simulink model "nms_sim_2D_cost"  (R2024b)
settings: Solver=ode15s  StartTime=0.0  StopTime=t_sim  MaxStep=dt_max  EnableMultiTasking=on
values from neighbouring files (symbols this model uses):
  a_BFSH = param_ctrl(35)*1    [setCtrlPar_optim_CPGreflex2001_2D.m]
  a_GAS = param_ctrl(37)*1    [setCtrlPar_optim_CPGreflex2001_2D.m]
  a_GLU = param_ctrl(31)*1    [setCtrlPar_optim_CPGreflex2001_2D.m]
  a_HAM = param_ctrl(33)*1    [setCtrlPar_optim_CPGreflex2001_2D.m]
  a_HFL = param_ctrl(32)*1    [setCtrlPar_optim_CPGreflex2001_2D.m]
  a_RF = param_ctrl(34)*1    [setCtrlPar_optim_CPGreflex2001_2D.m]
  a_SOL = param_ctrl(38)*1    [setCtrlPar_optim_CPGreflex2001_2D.m]
  a_TA = param_ctrl(39)*1    [setCtrlPar_optim_CPGreflex2001_2D.m]
  a_VAS = param_ctrl(36)*1    [setCtrlPar_optim_CPGreflex2001_2D.m]
  ai = param_ctrl(96)*2.0    [setCtrlPar_optim_CPGreflex2001_2D.m]
  b_BFSH = param_ctrl(52)*.51    [setCtrlPar_optim_CPGreflex2001_2D.m]
  b_BFSHGAS = param_ctrl(55)*.51    [setCtrlPar_optim_CPGreflex2001_2D.m]
  b_BFSHHAM = param_ctrl(54)*.51    [setCtrlPar_optim_CPGreflex2001_2D.m]
  b_BFSHVAS = param_ctrl(53)*.51    [setCtrlPar_optim_CPGreflex2001_2D.m]
  b_GAS = param_ctrl(59)*.51    [setCtrlPar_optim_CPGreflex2001_2D.m]
  b_GASBFSH = param_ctrl(60)*.51    [setCtrlPar_optim_CPGreflex2001_2D.m]
  b_GASSOL = param_ctrl(61)*.51    [setCtrlPar_optim_CPGreflex2001_2D.m]
  b_GLU = param_ctrl(40)*.51    [setCtrlPar_optim_CPGreflex2001_2D.m]
  b_GLUHAM = param_ctrl(42)*.51    [setCtrlPar_optim_CPGreflex2001_2D.m]
  b_GLUHFL = param_ctrl(41)*.51    [setCtrlPar_optim_CPGreflex2001_2D.m]
  b_HAM = param_ctrl(46)*.51    [setCtrlPar_optim_CPGreflex2001_2D.m]
  b_HAMBFSH = param_ctrl(48)*.51    [setCtrlPar_optim_CPGreflex2001_2D.m]
  b_HAMGLU = param_ctrl(47)*.51    [setCtrlPar_optim_CPGreflex2001_2D.m]
  b_HFL = param_ctrl(43)*.51    [setCtrlPar_optim_CPGreflex2001_2D.m]
  b_HFLGLU = param_ctrl(44)*.51    [setCtrlPar_optim_CPGreflex2001_2D.m]
  b_HFLRF = param_ctrl(45)*.51    [setCtrlPar_optim_CPGreflex2001_2D.m]
  b_RF = param_ctrl(49)*.51    [setCtrlPar_optim_CPGreflex2001_2D.m]
  b_RFHFL = param_ctrl(50)*.51    [setCtrlPar_optim_CPGreflex2001_2D.m]
  b_RFVAS = param_ctrl(51)*.51    [setCtrlPar_optim_CPGreflex2001_2D.m]
  b_SOL = param_ctrl(62)*.51    [setCtrlPar_optim_CPGreflex2001_2D.m]
  b_SOLGAS = param_ctrl(64)*.51    [setCtrlPar_optim_CPGreflex2001_2D.m]
  b_SOLTA = param_ctrl(63)*.51    [setCtrlPar_optim_CPGreflex2001_2D.m]
  b_TA = param_ctrl(65)*.51    [setCtrlPar_optim_CPGreflex2001_2D.m]
  b_TASOL = param_ctrl(66)*.51    [setCtrlPar_optim_CPGreflex2001_2D.m]
  b_VAS = param_ctrl(56)*.51    [setCtrlPar_optim_CPGreflex2001_2D.m]
  b_VASBFSH = param_ctrl(57)*.51    [setCtrlPar_optim_CPGreflex2001_2D.m]
  b_VASRF = param_ctrl(58)*.51    [setCtrlPar_optim_CPGreflex2001_2D.m]
  bias = param_ctrl(97)*2.5    [setCtrlPar_optim_CPGreflex2001_2D.m]
  c = 0.05    [nms_MS_2D_scaled.m]
  c_jointstop = 0.3 / (pi/180)    (= 17.1887338539)    [nms_MS_2D_scaled.m]
  D12_F = 0.16    *scaleL_JPhys    [nms_MechInit_2D_scaleSkel.m]
  D12_S = 0.2460	*sub_height    [nms_MechInit_2D_scaleSkel.m]
  D12_T = 0.2450  *sub_height    [nms_MechInit_2D_scaleSkel.m]
  D12y_F = 0.039  *sub_height    [nms_MechInit_2D_scaleSkel.m]
  D12z_HAT = 0.1    [nms_MS_2D_scaled.m]
  D13_F = 0.20    *scaleL_JPhys    [nms_MechInit_2D_scaleSkel.m]
  D1G_F = 0.14    *scaleL_JPhys    [nms_MechInit_2D_scaleSkel.m]
  D1G_HAT = 0.35  *scaleL_JPhys    [nms_MechInit_2D_scaleSkel.m]
  D1G_S = (0.3 - D12y_F/4)	*scaleL_JPhys    [nms_MechInit_2D_scaleSkel.m]
  D1G_T = (0.3 - D12y_F/4)	*scaleL_JPhys    [nms_MechInit_2D_scaleSkel.m]
  D1Gy_F = D12y_F*D1G_F/D12_F    (= 0.07)    [nms_MechInit_2D_scaleSkel.m]
  d_BFSH = param_ctrl(26)*1    [setCtrlPar_optim_CPGreflex2001_2D.m]
  d_GAS = param_ctrl(28)*1    [setCtrlPar_optim_CPGreflex2001_2D.m]
  d_GLU = param_ctrl(22)*1    [setCtrlPar_optim_CPGreflex2001_2D.m]
  d_HAM = param_ctrl(24)*1    [setCtrlPar_optim_CPGreflex2001_2D.m]
  d_HFL = param_ctrl(23)*1    [setCtrlPar_optim_CPGreflex2001_2D.m]
  d_RF = param_ctrl(25)*1    [setCtrlPar_optim_CPGreflex2001_2D.m]
  d_SOL = param_ctrl(29)*1    [setCtrlPar_optim_CPGreflex2001_2D.m]
  d_TA = param_ctrl(30)*1    [setCtrlPar_optim_CPGreflex2001_2D.m]
  d_VAS = param_ctrl(27)*1    [setCtrlPar_optim_CPGreflex2001_2D.m]
  DeltaThRef = 5e-3    (= 0.005)    [nms_MS_2D_scaled.m]
  dloptBFSH = 3.0    (= 3)    [setCtrlPar_optim_CPGreflex2001_2D.m]
  dloptGAS = 3.0    (= 3)    [setCtrlPar_optim_CPGreflex2001_2D.m]
  dloptGLU = 3.0    (= 3)    [setCtrlPar_optim_CPGreflex2001_2D.m]
  dloptHAM = 3.0    (= 3)    [setCtrlPar_optim_CPGreflex2001_2D.m]
  dloptHFL = 3.0    (= 3)    [setCtrlPar_optim_CPGreflex2001_2D.m]
  dloptRF = 3.0    (= 3)    [setCtrlPar_optim_CPGreflex2001_2D.m]
  dloptSOL = 3.0    (= 3)    [setCtrlPar_optim_CPGreflex2001_2D.m]
  dloptTA = 3.0    (= 3)    [setCtrlPar_optim_CPGreflex2001_2D.m]
  dloptVAS = 3.0    (= 3)    [setCtrlPar_optim_CPGreflex2001_2D.m]
  ec_BFSH = param_ctrl(80)*0.15    [setCtrlPar_optim_CPGreflex2001_2D.m]
  ec_GAS = param_ctrl(82)*0.15    [setCtrlPar_optim_CPGreflex2001_2D.m]
  ec_GLU = param_ctrl(76)*0.15    [setCtrlPar_optim_CPGreflex2001_2D.m]
  ec_HAM = param_ctrl(78)*0.15    [setCtrlPar_optim_CPGreflex2001_2D.m]
  ec_HFL = param_ctrl(77)*0.15    [setCtrlPar_optim_CPGreflex2001_2D.m]
  ec_RF = param_ctrl(79)*0.15    [setCtrlPar_optim_CPGreflex2001_2D.m]
  ec_TA = param_ctrl(84)*0.15    [setCtrlPar_optim_CPGreflex2001_2D.m]
  ec_VAS = param_ctrl(81)*0.15    [setCtrlPar_optim_CPGreflex2001_2D.m]
  eref = 0.04    [nms_MS_2D_scaled.m]
  eref_GAS = 0.1    [nms_MS_2D_scaled.m]
  eref_SOL = 0.1    [nms_MS_2D_scaled.m]
  es_BFSH = param_ctrl(89)*0.15    [setCtrlPar_optim_CPGreflex2001_2D.m]
  es_GAS = param_ctrl(91)*0.15    [setCtrlPar_optim_CPGreflex2001_2D.m]
  es_GLU = param_ctrl(85)*0.15    [setCtrlPar_optim_CPGreflex2001_2D.m]
  es_HAM = param_ctrl(87)*0.15    [setCtrlPar_optim_CPGreflex2001_2D.m]
  es_HFL = param_ctrl(86)*0.15    [setCtrlPar_optim_CPGreflex2001_2D.m]
  es_RF = param_ctrl(88)*0.15    [setCtrlPar_optim_CPGreflex2001_2D.m]
  es_TA = param_ctrl(93)*0.15    [setCtrlPar_optim_CPGreflex2001_2D.m]
  es_VAS = param_ctrl(90)*0.15    [setCtrlPar_optim_CPGreflex2001_2D.m]
  FmaxBFSH = 350    [nms_MS_2D_scaled.m]
  FmaxGAS = 2000    [nms_MS_2D_scaled.m]
  FmaxGLU = 4000    [nms_MS_2D_scaled.m]
  FmaxHAM = 2000    [nms_MS_2D_scaled.m]
  FmaxHFL = 2000    [nms_MS_2D_scaled.m]
  FmaxRF = 850    [nms_MS_2D_scaled.m]
  FmaxSOL = 4000    [nms_MS_2D_scaled.m]
  FmaxTA = 800    [nms_MS_2D_scaled.m]
  FmaxVAS = 5000    [nms_MS_2D_scaled.m]
  g = 9.81    [nms_MS_2D_scaled.m]
  gamma_4 = param_ctrl(11) * 1.7    [setCtrlPar_optim_CPGreflexsynergy2023_2D.m]
  h_BFSH = param_ctrl(71)*.1    [setCtrlPar_optim_CPGreflex2001_2D.m]
  h_GAS = param_ctrl(73)*.1    [setCtrlPar_optim_CPGreflex2001_2D.m]
  h_GLU = param_ctrl(67)*.1    [setCtrlPar_optim_CPGreflex2001_2D.m]
  h_HAM = param_ctrl(69)*.1    [setCtrlPar_optim_CPGreflex2001_2D.m]
  h_HFL = param_ctrl(68)*.1    [setCtrlPar_optim_CPGreflex2001_2D.m]
  h_RF = param_ctrl(70)*.1    [setCtrlPar_optim_CPGreflex2001_2D.m]
  h_SOL = param_ctrl(74)*.1    [setCtrlPar_optim_CPGreflex2001_2D.m]
  h_TA = param_ctrl(75)*.1    [setCtrlPar_optim_CPGreflex2001_2D.m]
  h_VAS = param_ctrl(72)*.1    [setCtrlPar_optim_CPGreflex2001_2D.m]
  HLCtrlPar = [theta_tgt l_clr alpha_tgt alpha_cd alpha_cv]    [setCtrlPar_optim_reflex2015_2D.m]
  In_F = 0.005    *scaleM*scaleL_JPhys^2    [nms_MechInit_2D_scaleSkel.m]
  In_HAT = 2.5    *scaleM*scaleL_JPhys^2    [nms_MechInit_2D_scaleSkel.m]
  In_S = 0.05     *scaleM*scaleL_JPhys^2    [nms_MechInit_2D_scaleSkel.m]
  In_T = 0.15     *scaleM*scaleL_JPhys^2    [nms_MechInit_2D_scaleSkel.m]
  init_exc = 0.01    [setInitPar_optim_2D.m]
  init_fm = 0.01    [setInitPar_optim_2D.m]
  init_lce = 1    [setInitPar_optim_2D.m]
  init_LCPG = param_ctrl(12) * 0.01    [setCtrlPar_optim_CPGreflexsynergy2023_2D.m]
  init_LStance = 1    [setInitPar_optim_2D.m]
  init_N1 = osc_signal1(phi_off_osc_ind)    [setCtrlPar_optim_CPGreflex2001_2D.m]
  ... (+441 more)
undefined symbols (not defined in the file or in its folder): cost_act_exponent, cost_v_tgt, flag_controller, Newton, nStep_obj, nStep_startKin, Raphson, sgn, SSW_kin, terrain_slope_angle, v_plateS1, X, Y, Z
libraries: nesl_utility x94, sm_lib x90, simulink x28, simulink_extras x12
(part 9 of 20)

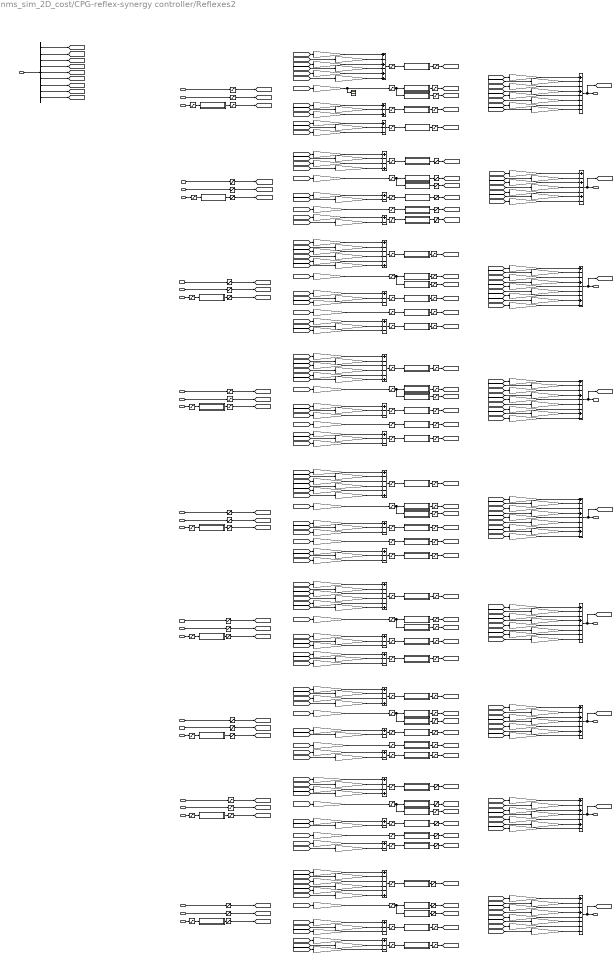
== system nms_sim_2D_cost/CPG-reflex-synergy controller/Reflexes2 ==
  note: GLU
  note: Sensory Neurons
  note: Inter Neurons
  note: Reflex output to Motoneurons
  note: HFL
  note: HAM
  note: RF
  note: VAS
  note: BFSH
  note: GAS
  note: SOL
  note: TA
  note: Muscle Activations (MN) RC
  FmGLU : Inport
  LceGLU : Inport  Port=2
  VceGLU : Inport  Port=3
  FmHFL : Inport  Port=4
  LceHFL : Inport  Port=5
  VceHFL : Inport  Port=6
  FmHAM : Inport  Port=7
  LceHAM : Inport  Port=8
  VceHAM : Inport  Port=9
  FmRF : Inport  Port=10
  LceRF : Inport  Port=11
  VceRF : Inport  Port=12
  FmVAS : Inport  Port=13
  LceVAS : Inport  Port=14
  VceVAS : Inport  Port=15
  FmBFSH : Inport  Port=16
  LceBFSH : Inport  Port=17
  VceBFSH : Inport  Port=18
  FmGAS : Inport  Port=19
  LceGAS : Inport  Port=20
  VceGAS : Inport  Port=21
  FmSOL : Inport  Port=22
  LceSOL : Inport  Port=23
  VceSOL : Inport  Port=24
  FmTA : Inport  Port=25
  LceTA : Inport  Port=26
  VceTA : Inport  Port=27
  Act : Inport  Port=28
  Demux : Demux  Outputs=9
  Gain1 : Gain  Gain=k_INIA_HFL_SNIA_HFL
  Gain10 : Gain  Gain=k_INIB_HFL_INIB_HAM
  Gain100 : Gain  Gain=k_INIA_TA_INIA_GAS
  Gain101 : Gain  Gain=k_INIA_TA_INIA_SOL
  Gain102 : Gain  Gain=k_INIA_TA_INRC_GAS
  Gain103 : Gain  Gain=k_INIA_TA_INRC_SOL
  Gain104 : Gain  Gain=k_INIA_TA_MN_TA
  Gain105 : Gain  Gain=k_INII_TA_SNII_TA
  Gain106 : Gain  Gain=k_INIB_TA_SNIB_TA
  Gain107 : Gain  Gain=k_INIB_TA_INIB_GAS
  Gain108 : Gain  Gain=k_INIB_TA_INIB_SOL
  Gain109 : Gain  Gain=k_INRC_TA_Act_TA
  Gain11 : Gain  Gain=k_INRC_HFL_INRC_HAM
  Gain110 : Gain  Gain=k_INRC_TA_INRC_GAS
  Gain111 : Gain  Gain=k_INRC_TA_INRC_SOL
  Gain112 : Gain  Gain=k_MN_HFL_SNIA_HFL
  Gain113 : Gain  Gain=k_MN_HFL_INIA_GLU
  Gain114 : Gain  Gain=k_MN_HFL_INIA_HAM
  Gain115 : Gain  Gain=k_MN_HFL_INII_HFL
  Gain116 : Gain  Gain=k_MN_HFL_INII_GLU
  Gain117 : Gain  Gain=k_MN_HFL_INII_HAM
  Gain118 : Gain  Gain=k_MN_HFL_INIB_HFL
  Gain119 : Gain  Gain=k_MN_HFL_INRC_HFL
  Gain12 : Gain  Gain=k_INRC_HFL_Act_HFL
  Gain120 : Gain  Gain=k_MN_GLU_SNIA_GLU
  Gain121 : Gain  Gain=k_MN_GLU_INIA_HFL
  Gain122 : Gain  Gain=k_MN_GLU_INII_GLU
  Gain123 : Gain  Gain=k_MN_GLU_INII_HFL
  Gain124 : Gain  Gain=k_MN_GLU_INIB_GLU
  Gain125 : Gain  Gain=k_MN_GLU_INIBext_GLU
  Gain126 : Gain  Gain=k_MN_GLU_INRC_GLU
  Gain127 : Gain  Gain=k_MN_HAM_SNIA_HAM
  Gain128 : Gain  Gain=k_MN_HAM_INIA_VAS
  Gain129 : Gain  Gain=k_MN_HAM_INIA_RF
  Gain13 : Gain  Gain=k_INRC_HFL_INRC_GLU
  Gain130 : Gain  Gain=k_MN_HAM_INII_HAM
  Gain131 : Gain  Gain=k_MN_HAM_INII_VAS
  Gain132 : Gain  Gain=k_MN_HAM_INII_RF
  Gain133 : Gain  Gain=k_MN_HAM_INIB_HAM
  Gain134 : Gain  Gain=k_MN_HAM_INIBext_HAM
  Gain135 : Gain  Gain=k_MN_HAM_INRC_HAM
  Gain136 : Gain  Gain=k_MN_RF_SNIA_RF
  Gain137 : Gain  Gain=k_MN_RF_INIA_HAM
  Gain138 : Gain  Gain=k_MN_RF_INIA_BFSH
  Gain139 : Gain  Gain=k_MN_RF_INII_RF
  Gain14 : Gain  Gain=k_INIA_GLU_INRC_HFL
  Gain140 : Gain  Gain=k_MN_RF_INII_HAM
  Gain141 : Gain  Gain=k_MN_RF_INII_BFSH
  Gain142 : Gain  Gain=k_MN_RF_INIB_RF
  Gain143 : Gain  Gain=k_MN_RF_INIBext_RF
  Gain144 : Gain  Gain=k_MN_RF_INRC_RF
  Gain145 : Gain  Gain=k_MN_VAS_SNIA_VAS
  Gain146 : Gain  Gain=k_MN_VAS_INIA_HAM
  Gain147 : Gain  Gain=k_MN_VAS_INIA_BFSH
  Gain148 : Gain  Gain=k_MN_VAS_INII_VAS
  Gain149 : Gain  Gain=k_MN_VAS_INII_HAM
  Gain15 : Gain  Gain=k_INIA_GLU_SNIA_GLU
  Gain150 : Gain  Gain=k_MN_VAS_INII_BFSH
  Gain151 : Gain  Gain=k_MN_VAS_INIB_VAS
  Gain152 : Gain  Gain=k_MN_VAS_INIBext_VAS
  Gain153 : Gain  Gain=k_MN_VAS_INRC_VAS
  Gain154 : Gain  Gain=k_MN_BFSH_SNIA_BFSH
  Gain155 : Gain  Gain=k_MN_BFSH_INIA_VAS
  Gain156 : Gain  Gain=k_MN_BFSH_INIA_RF
  Gain157 : Gain  Gain=k_MN_BFSH_INII_BFSH
  Gain158 : Gain  Gain=k_MN_BFSH_INII_VAS
  Gain159 : Gain  Gain=k_MN_BFSH_INII_RF
  Gain16 : Gain  Gain=k_INIA_GLU_INIA_HFL
  Gain160 : Gain  Gain=k_MN_BFSH_INIB_BFSH
  Gain161 : Gain  Gain=k_MN_BFSH_INRC_BFSH
  Gain162 : Gain  Gain=k_MN_GAS_SNIA_GAS
  Gain163 : Gain  Gain=k_MN_GAS_INIA_TA
  Gain164 : Gain  Gain=k_MN_GAS_INII_GAS
  Gain165 : Gain  Gain=k_MN_GAS_INII_TA
  Gain166 : Gain  Gain=k_MN_GAS_INIB_GAS
  Gain167 : Gain  Gain=k_MN_GAS_INIBext_GAS
  Gain168 : Gain  Gain=k_MN_GAS_INRC_GAS
  Gain169 : Gain  Gain=k_MN_SOL_SNIA_SOL
  Gain17 : Gain  Gain=k_INIA_GLU_MN_GLU
  Gain170 : Gain  Gain=k_MN_SOL_INIA_TA
  Gain171 : Gain  Gain=k_MN_SOL_INII_SOL
  Gain172 : Gain  Gain=k_MN_SOL_INII_TA
  Gain173 : Gain  Gain=k_MN_SOL_INIB_SOL
  Gain174 : Gain  Gain=k_MN_SOL_INIBext_SOL
  Gain175 : Gain  Gain=k_MN_SOL_INRC_SOL
  Gain176 : Gain  Gain=k_MN_TA_SNIA_TA
  Gain177 : Gain  Gain=k_MN_TA_INIA_GAS
  Gain178 : Gain  Gain=k_MN_TA_INIA_SOL
  Gain179 : Gain  Gain=k_MN_TA_INII_TA
  Gain18 : Gain  Gain=k_INII_GLU_SNII_GLU
  Gain180 : Gain  Gain=k_MN_TA_INII_GAS
  Gain181 : Gain  Gain=k_MN_TA_INII_SOL
  Gain182 : Gain  Gain=k_MN_TA_INIB_TA
  Gain183 : Gain  Gain=k_MN_TA_INRC_TA
  Gain19 : Gain  Gain=k_INIB_GLU_SNIB_GLU
  Gain2 : Gain  Gain=k_INIA_HFL_INIA_GLU
  Gain20 : Gain  Gain=k_INIB_GLU_INIB_HFL
  Gain21 : Gain  Gain=k_INIB_GLU_SNIBext_GLU
  Gain22 : Gain  Gain=k_INRC_GLU_Act_GLU
  Gain23 : Gain  Gain=k_INRC_GLU_INRC_HFL
  Gain24 : Gain  Gain=k_INIA_HAM_SNIA_HAM
  Gain25 : Gain  Gain=k_INIA_HAM_INIA_VAS
  Gain26 : Gain  Gain=k_INIA_HAM_INIA_RF
  Gain27 : Gain  Gain=k_INIA_HAM_INRC_VAS
  Gain28 : Gain  Gain=k_INIA_HAM_INRC_RF
  Gain29 : Gain  Gain=k_INIA_HAM_MN_HAM
  Gain3 : Gain  Gain=k_INIA_HFL_INIA_HAM
  Gain30 : Gain  Gain=k_INII_HAM_SNII_HAM
  Gain31 : Gain  Gain=k_INIB_HAM_SNIB_HAM
  Gain32 : Gain  Gain=k_INIB_HAM_INIB_VAS
  Gain33 : Gain  Gain=k_INIB_HAM_INIB_RF
  Gain34 : Gain  Gain=k_INIB_HAM_SNIBext_HAM
  Gain35 : Gain  Gain=k_INRC_HAM_Act_HAM
  Gain36 : Gain  Gain=k_INRC_HAM_INRC_VAS
  Gain37 : Gain  Gain=k_INRC_HAM_INRC_RF
  Gain38 : Gain  Gain=k_INIA_RF_SNIA_RF
  Gain39 : Gain  Gain=k_INIA_RF_INIA_HAM
  Gain4 : Gain  Gain=k_INIA_HFL_INRC_GLU
  Gain40 : Gain  Gain=k_INIA_RF_INIA_BFSH
  Gain41 : Gain  Gain=k_INIA_RF_INRC_HAM
  Gain42 : Gain  Gain=k_INIA_RF_INRC_BFSH
  Gain43 : Gain  Gain=k_INIA_RF_MN_RF
  Gain44 : Gain  Gain=k_INII_RF_SNII_RF
  Gain45 : Gain  Gain=k_INIB_RF_SNIB_RF
  Gain46 : Gain  Gain=k_INIB_RF_INIB_HAM
  Gain47 : Gain  Gain=k_INIB_RF_INIB_BFSH
  Gain48 : Gain  Gain=k_INIB_RF_SNIBext_RF
  Gain49 : Gain  Gain=k_INRC_RF_Act_RF
  Gain5 : Gain  Gain=k_INIA_HFL_INRC_HAM
  Gain50 : Gain  Gain=k_INRC_RF_INRC_HAM
  Gain51 : Gain  Gain=k_INRC_RF_INRC_BFSH
  Gain52 : Gain  Gain=k_INIA_VAS_SNIA_VAS
  Gain53 : Gain  Gain=k_INIA_VAS_INIA_HAM
  Gain54 : Gain  Gain=k_INIA_VAS_INIA_BFSH
  Gain55 : Gain  Gain=k_INIA_VAS_INRC_HAM
  Gain56 : Gain  Gain=k_INIA_VAS_INRC_BFSH
  Gain57 : Gain  Gain=k_INIA_VAS_MN_VAS
  Gain58 : Gain  Gain=k_INII_VAS_SNII_VAS
  Gain59 : Gain  Gain=k_INIB_VAS_SNIB_VAS
  Gain6 : Gain  Gain=k_INII_HFL_SNII_HFL
  Gain60 : Gain  Gain=k_INIB_VAS_INIB_HAM
  Gain61 : Gain  Gain=k_INIB_VAS_INIB_BFSH
  Gain62 : Gain  Gain=k_INRC_VAS_Act_VAS
  Gain63 : Gain  Gain=k_INRC_VAS_INRC_HAM
  Gain64 : Gain  Gain=k_INRC_VAS_INRC_BFSH
  Gain65 : Gain  Gain=k_INIB_VAS_SNIBext_VAS
  Gain66 : Gain  Gain=k_INIA_BFSH_SNIA_BFSH
  Gain67 : Gain  Gain=k_INIA_BFSH_INIA_VAS
  Gain68 : Gain  Gain=k_INIA_BFSH_INIA_RF
  Gain69 : Gain  Gain=k_INIA_BFSH_INRC_VAS
  Gain7 : Gain  Gain=k_INIA_HFL_MN_HFL
  Gain70 : Gain  Gain=k_INIA_BFSH_INRC_RF
  Gain71 : Gain  Gain=k_INIA_BFSH_MN_BFSH
  Gain72 : Gain  Gain=k_INII_BFSH_SNII_BFSH
  Gain73 : Gain  Gain=k_INIB_BFSH_SNIB_BFSH
  Gain74 : Gain  Gain=k_INIB_BFSH_INIB_VAS
  Gain75 : Gain  Gain=k_INIB_BFSH_INIB_RF
  Gain76 : Gain  Gain=k_INRC_BFSH_Act_BFSH
  Gain77 : Gain  Gain=k_INRC_BFSH_INRC_VAS
  Gain78 : Gain  Gain=k_INRC_BFSH_INRC_RF
  Gain79 : Gain  Gain=k_INIA_GAS_SNIA_GAS
  Gain8 : Gain  Gain=k_INIB_HFL_SNIB_HFL
  Gain80 : Gain  Gain=k_INIA_GAS_INIA_TA
  Gain81 : Gain  Gain=k_INIA_GAS_INRC_TA
  Gain82 : Gain  Gain=k_INIA_GAS_MN_GAS
  Gain83 : Gain  Gain=k_INII_GAS_SNII_GAS
  Gain84 : Gain  Gain=k_INIB_GAS_SNIB_GAS
  Gain85 : Gain  Gain=k_INIB_GAS_INIB_TA
  Gain86 : Gain  Gain=k_INRC_GAS_Act_GAS
  Gain87 : Gain  Gain=k_INRC_GAS_INRC_TA
  Gain88 : Gain  Gain=k_INIB_GAS_SNIBext_GAS
  Gain89 : Gain  Gain=k_INIA_SOL_SNIA_SOL
  Gain9 : Gain  Gain=k_INIB_HFL_INIB_GLU
  Gain90 : Gain  Gain=k_INIA_SOL_INIA_TA
  Gain91 : Gain  Gain=k_INIA_SOL_INRC_TA
  Gain92 : Gain  Gain=k_INIA_SOL_MN_SOL
  Gain93 : Gain  Gain=k_INII_SOL_SNII_SOL
  Gain94 : Gain  Gain=k_INIB_SOL_SNIB_SOL
  Gain95 : Gain  Gain=k_INIB_SOL_INIB_TA
  Gain96 : Gain  Gain=k_INIB_SOL_SNIBext_SOL
  Gain97 : Gain  Gain=k_INRC_SOL_Act_SOL
  Gain98 : Gain  Gain=k_INRC_SOL_INRC_TA
  Gain99 : Gain  Gain=k_INIA_TA_SNIA_TA
  IN RC1 : Subsystem
  IN RC10 : Subsystem
  IN RC11 : Subsystem
  IN RC12 : Subsystem
  IN RC13 : Subsystem
  IN RC14 : Subsystem
  IN RC15 : Subsystem
  IN RC16 : Subsystem
  IN RC17 : Subsystem
  IN RC18 : Subsystem
  IN RC19 : Subsystem
  IN RC2 : Subsystem
  IN RC20 : Subsystem
  IN RC21 : Subsystem
  IN RC22 : Subsystem
  IN RC23 : Subsystem
  IN RC24 : Subsystem
  IN RC25 : Subsystem
  IN RC26 : Subsystem
  IN RC27 : Subsystem
  IN RC28 : Subsystem
  IN RC29 : Subsystem
  IN RC3 : Subsystem
  IN RC30 : Subsystem
  IN RC31 : Subsystem
  IN RC32 : Subsystem
  IN RC33 : Subsystem
  IN RC34 : Subsystem
  IN RC35 : Subsystem
  IN RC36 : Subsystem
  IN RC37 : Subsystem
  IN RC38 : Subsystem
  IN RC39 : Subsystem
  IN RC4 : Subsystem
  IN RC40 : Subsystem
  IN RC41 : Subsystem
  IN RC42 : Subsystem
  IN RC43 : Subsystem
  IN RC44 : Subsystem
  IN RC45 : Subsystem
  IN RC46 : Subsystem
  IN RC47 : Subsystem
  IN RC48 : Subsystem
  IN RC49 : Subsystem
  IN RC5 : Subsystem
  IN RC50 : Subsystem
  IN RC51 : Subsystem
  IN RC6 : Subsystem
  IN RC7 : Subsystem
  IN RC8 : Subsystem
  IN RC9 : Subsystem
  SN : Subsystem
  SN1 : Subsystem
  SN2 : Subsystem
  SN3 : Subsystem
  SN4 : Subsystem
  SN5 : Subsystem
  SN6 : Subsystem
  SN7 : Subsystem
  SN8 : Subsystem
  Saturation{,1..8,51..77} (36 alike) : Saturate  UpperLimit=inf  LowerLimit=0
  Saturation{9..50,78..86} (51 alike) : Saturate  UpperLimit=1  LowerLimit=0.01
  Saturation{87..128} (42 alike) : Saturate  UpperLimit=2  LowerLimit=-2
  Scope20 : Scope
  Sum : Sum  Inputs=+--+
  Sum1 : Sum  Inputs=+-+-++
  Sum{5,7..8,10..13,16..17,25..26} (11 alike) : Sum  Inputs=+--
  Sum{6,9,14..15,24} (5 alike) : Sum  Inputs=+----+
  Sum18 : Sum  Inputs=+--+
  Sum{2..3,19..20,22..23} (6 alike) : Sum  Inputs=+-
  Sum21 : Sum  Inputs=+--+
  Sum27 : Sum  Inputs=+-+--+-
  Sum28 : Sum  Inputs=+--+----
  Sum29 : Sum  Inputs=+--+---+-
  Sum30 : Sum  Inputs=+--+---+-
  Sum31 : Sum  Inputs=+--+---+-
  Sum32 : Sum  Inputs=+--+----
  Sum33 : Sum  Inputs=+-+--+-
  Sum34 : Sum  Inputs=+-+--+-
  Sum35 : Sum  Inputs=+--+----
  Sum4 : Sum  Inputs=+-+
  Outport : Outport
  Outport1 : Outport  Port=2
  Outport2 : Outport  Port=3
  Outport3 : Outport  Port=4
  Outport4 : Outport  Port=5
  Outport5 : Outport  Port=6
  Outport6 : Outport  Port=7
  Outport7 : Outport  Port=8
  Outport8 : Outport  Port=9
  wires:
  VceGLU/1 -> Saturation/1
  Saturation/1 -> SN/1(In1)
  SN1/1(Out1) -> Saturation53/1
  VceHAM/1 -> Saturation1/1
  SN/1(Out1) -> Saturation56/1
  VceHFL/1 -> Saturation2/1
  Saturation2/1 -> SN1/1(In1)
  Saturation1/1 -> SN2/1(In1)
  SN2/1(Out1) -> Saturation59/1
  LceGLU/1 -> Saturation55/1
  FmGLU/1 -> Saturation54/1
  FmHFL/1 -> Saturation51/1
  LceHFL/1 -> Saturation52/1
  FmHAM/1 -> Saturation57/1
  LceHAM/1 -> Saturation58/1
  [SN_IA_GLU] -> Gain15/1
  [IN_IA_HFL] -> Gain16/1
  IN RC42/1(out) -> Saturation13/1  "INIA GLU"
  IN RC48/1(out) -> Saturation9/1  "INIA HFL"
  LceRF/1 -> Saturation61/1
  FmRF/1 -> Saturation60/1
  SN3/1(Out1) -> Saturation62/1
  Saturation3/1 -> SN3/1(In1)
  VceRF/1 -> Saturation3/1
  Saturation4/1 -> SN4/1(In1)
  SN4/1(Out1) -> Saturation65/1
  FmVAS/1 -> Saturation63/1
  LceVAS/1 -> Saturation64/1
  [IN_RC_HFL] -> Gain14/1
  VceVAS/1 -> Saturation4/1
  VceBFSH/1 -> Saturation5/1
  LceBFSH/1 -> Saturation67/1
  FmBFSH/1 -> Saturation66/1
  SN5/1(Out1) -> Saturation68/1
  Saturation5/1 -> SN5/1(In1)
  Saturation6/1 -> SN6/1(In1)
  SN6/1(Out1) -> Saturation71/1
  FmGAS/1 -> Saturation69/1
  LceGAS/1 -> Saturation70/1
  VceGAS/1 -> Saturation6/1
  VceSOL/1 -> Saturation7/1
  LceSOL/1 -> Saturation73/1
  FmSOL/1 -> Saturation72/1
  SN7/1(Out1) -> Saturation74/1
  Saturation7/1 -> SN7/1(In1)
  Saturation8/1 -> SN8/1(In1)
  SN8/1(Out1) -> Saturation77/1
  FmTA/1 -> Saturation75/1
  LceTA/1 -> Saturation76/1
  VceTA/1 -> Saturation8/1
  [SN_II_GLU] -> Gain18/1
  IN RC43/1(out) -> Saturation14/1  "INII GLU1"
  IN RC44/1(out) -> Saturation85/1  "INII GLU2"
  IN RC45/1(out) -> Saturation15/1  "INIB GLU"
  [SN_IB_GLU] -> Gain19/1
  [IN_IB_HFL] -> Gain20/1
  [SN_IB_GLU] -> Gain21/1
  IN RC46/1(out) -> Saturation16/1  "INIBext GLU"
  IN RC47/1(out) -> Saturation17/1  "INRC GLU"
  [IN_RC_HFL] -> Gain23/1
  [Act_GLU] -> Gain22/1
  IN RC49/1(out) -> Saturation10/1  "INII HFL1"
  IN RC50/1(out) -> Saturation86/1  "INII HFL2"
  [SN_II_HFL] -> Gain6/1
  IN RC51/1(out) -> Saturation11/1  "INIB HFL"
  IN RC41/1(out) -> Saturation12/1  "INRC HFL"
  [IN_RC_RF] -> Gain28/1
  [SN_IA_HAM] -> Gain24/1
  [IN_IA_VAS] -> Gain25/1
  IN RC35/1(out) -> Saturation18/1
  [IN_RC_VAS] -> Gain27/1
  [IN_IA_RF] -> Gain26/1
  [IN_IB_RF] -> Gain33/1
  [SN_II_HAM] -> Gain30/1
  IN RC40/1(out) -> Saturation22/1
  IN RC37/1(out) -> Saturation84/1
  IN RC36/1(out) -> Saturation19/1
  IN RC38/1(out) -> Saturation20/1
  [SN_IB_HAM] -> Gain31/1
  [IN_IB_VAS] -> Gain32/1
  [IN_RC_RF] -> Gain37/1
  [IN_RC_VAS] -> Gain36/1
  IN RC39/1(out) -> Saturation21/1
  [SN_IB_HAM] -> Gain34/1
  [IN_RC_BFSH] -> Gain42/1
  IN RC29/1(out) -> Saturation23/1
  [IN_IA_BFSH] -> Gain40/1
  [SN_IA_RF] -> Gain38/1
  [IN_IA_HAM] -> Gain39/1
  [IN_RC_HAM] -> Gain41/1
  [SN_IB_RF] -> Gain45/1
  [IN_RC_BFSH] -> Gain51/1
  [SN_II_RF] -> Gain44/1
  IN RC30/1(out) -> Saturation24/1
  IN RC31/1(out) -> Saturation83/1
  IN RC34/1(out) -> Saturation27/1
  [SN_IB_RF] -> Gain48/1
  IN RC33/1(out) -> Saturation26/1
  [IN_IB_HAM] -> Gain46/1
  IN RC32/1(out) -> Saturation25/1
  [IN_IB_BFSH] -> Gain47/1
  [IN_RC_HAM] -> Gain50/1
  IN RC27/1(out) -> Saturation31/1
  [IN_IB_BFSH] -> Gain61/1
  IN RC26/1(out) -> Saturation30/1
  [SN_IB_VAS] -> Gain65/1
  IN RC24/1(out) -> Saturation29/1
  IN RC28/1(out) -> Saturation32/1
  IN RC25/1(out) -> Saturation82/1
  [IN_RC_HAM] -> Gain63/1
  [IN_IB_HAM] -> Gain60/1
  [SN_II_VAS] -> Gain58/1
  [IN_RC_BFSH] -> Gain56/1
  [SN_IA_VAS] -> Gain52/1
  [IN_RC_BFSH] -> Gain64/1
  [IN_IA_HAM] -> Gain53/1
  [IN_RC_HAM] -> Gain55/1
  [IN_IA_BFSH] -> Gain54/1
  IN RC23/1(out) -> Saturation28/1
  [SN_IB_VAS] -> Gain59/1
  [IN_IB_RF] -> Gain75/1
  [SN_II_BFSH] -> Gain72/1
  IN RC22/1(out) -> Saturation36/1
  IN RC20/1(out) -> Saturation81/1
  [SN_IB_BFSH] -> Gain73/1
  [IN_IA_RF] -> Gain68/1
  [IN_RC_VAS] -> Gain77/1
  [IN_RC_RF] -> Gain70/1
  IN RC19/1(out) -> Saturation34/1
  [SN_IA_BFSH] -> Gain66/1
  [IN_IA_VAS] -> Gain67/1
  [IN_RC_RF] -> Gain78/1
  [IN_IB_VAS] -> Gain74/1
  IN RC18/1(out) -> Saturation33/1
  [IN_RC_VAS] -> Gain69/1
  IN RC21/1(out) -> Saturation35/1
  IN RC16/1(out) -> Saturation40/1  "INIBEXT GAS"
  [SN_II_GAS] -> Gain83/1
  [SN_IB_GAS] -> Gain84/1
  IN RC15/1(out) -> Saturation39/1  "INIB GAS"
  IN RC14/1(out) -> Saturation79/1  "INII GAS  2"
  IN RC13/1(out) -> Saturation38/1  "INII GAS 1"
  IN RC17/1(out) -> Saturation41/1  "INRC GAS"
  [IN_RC_TA] -> Gain87/1
  [SN_IB_GAS] -> Gain88/1
  [SN_IA_GAS] -> Gain79/1
  IN RC12/1(out) -> Saturation37/1  "INIA GAS"
  [IN_IB_TA] -> Gain85/1
  [IN_RC_TA] -> Gain81/1
  [IN_IA_TA] -> Gain80/1
  [IN_RC_TA] -> Gain91/1
  IN RC6/1(out) -> Saturation43/1  "INII SOL 1"
  IN RC7/1(out) -> Saturation80/1  "INII SOL 2"
  [IN_IB_TA] -> Gain95/1
  [SN_IB_SOL] -> Gain96/1
  [IN_IA_TA] -> Gain90/1
  IN RC5/1(out) -> Saturation42/1  "INIA SOL"
  IN RC11/1(out) -> Saturation46/1  "INRC SOL"
  [SN_IA_SOL] -> Gain89/1
  [IN_RC_TA] -> Gain98/1
  IN RC9/1(out) -> Saturation44/1  "INIB SOL"
  [SN_IB_SOL] -> Gain94/1
  IN RC10/1(out) -> Saturation45/1  "INIB EXT SOL"
  [SN_II_SOL] -> Gain93/1
  [IN_IB_SOL] -> Gain108/1
  [SN_II_TA] -> Gain105/1
  IN RC8/1(out) -> Saturation78/1  "INRC TA"
  IN RC2/1(out) -> Saturation49/1  "INII TA 2"
  [SN_IB_TA] -> Gain106/1
  [IN_IA_SOL] -> Gain101/1
  [IN_RC_GAS] -> Gain110/1
  [IN_RC_SOL] -> Gain103/1
  IN RC3/1(out) -> Saturation48/1  "INII TA 1"
  [SN_IA_TA] -> Gain99/1
  [IN_IA_GAS] -> Gain100/1
  [IN_RC_SOL] -> Gain111/1
  [IN_IB_GAS] -> Gain107/1
  IN RC4/1(out) -> Saturation47/1  "INIA TA"
  [IN_RC_GAS] -> Gain102/1
  IN RC1/1(out) -> Saturation50/1  "INIB TA"
  Demux/1 -> [Act_HFL]
  Demux/9 -> [Act_TA]
  Demux/8 -> [Act_SOL]
  Demux/7 -> [Act_GAS]
  Demux/6 -> [Act_BFSH]
  Demux/5 -> [Act_VAS]
  Demux/4 -> [Act_RF]
  Demux/3 -> [Act_HAM]
  Demux/2 -> [Act_GLU]
  Act/1 -> Demux/1
  [Act_HAM] -> Gain35/1
  [Act_RF] -> Gain49/1
  [Act_VAS] -> Gain62/1
  [Act_BFSH] -> Gain76/1
  [Act_GAS] -> Gain86/1
  [Act_SOL] -> Gain97/1
  [Act_TA] -> Gain109/1
  [IN_RC_GLU] -> Gain126/1
  [IN_IBext_GLU] -> Gain125/1
  [IN_IB_GLU] -> Gain124/1
  [IN_II_HFL_1] -> Gain123/1
  [IN_II_GLU_2] -> Gain122/1
  [IN_IA_HFL] -> Gain121/1
  [SN_IA_GLU] -> Gain120/1
  Sum27/1 -> [MN_GLU], Outport/1
  [MN_GLU] -> Gain17/1
  [MN_HAM] -> Gain29/1
  [MN_RF] -> Gain43/1
  [MN_VAS] -> Gain57/1
  [MN_BFSH] -> Gain71/1
  [MN_GAS] -> Gain82/1
  [MN_SOL] -> Gain92/1
  [MN_TA] -> Gain104/1
  [SN_IA_HFL] -> Gain112/1
  [IN_IA_GLU] -> Gain113/1
  [IN_IA_HAM] -> Gain114/1
  [IN_II_HFL_2] -> Gain115/1
  [IN_II_GLU_1] -> Gain116/1
  [IN_II_HAM_1] -> Gain117/1
  [IN_IB_HFL] -> Gain118/1
  [IN_RC_HFL] -> Gain119/1
  Sum28/1 -> Outport1/1, [MN_HFL]
  [IN_RC_HAM] -> Gain135/1
  [IN_IBext_HAM] -> Gain134/1
  [IN_IB_HAM] -> Gain133/1
  [IN_II_RF_1] -> Gain132/1
  [IN_II_VAS_1] -> Gain131/1
  [IN_II_HAM_2] -> Gain130/1
  [IN_IA_RF] -> Gain129/1
  [IN_IA_VAS] -> Gain128/1
  [SN_IA_HAM] -> Gain127/1
  Sum29/1 -> [MN_HAM], Outport2/1
  [IN_II_RF_2] -> Gain139/1
  [IN_II_HAM_1] -> Gain140/1
  [IN_IA_BFSH] -> Gain138/1
  [IN_IBext_RF] -> Gain143/1
  [SN_IA_RF] -> Gain136/1
  [IN_IA_HAM] -> Gain137/1
  [IN_RC_RF] -> Gain144/1
  [IN_IB_RF] -> Gain142/1
  Sum30/1 -> [MN_RF], Outport3/1
  [IN_II_BFSH_1] -> Gain141/1
  Sum31/1 -> [MN_VAS], Outport4/1
  [IN_II_BFSH_1] -> Gain150/1
  [IN_IA_BFSH] -> Gain147/1
  [IN_IA_HAM] -> Gain146/1
  [IN_II_HAM_1] -> Gain149/1
  [SN_IA_VAS] -> Gain145/1
  [IN_IB_VAS] -> Gain151/1
  [IN_II_VAS_2] -> Gain148/1
  [IN_IBext_VAS] -> Gain152/1
  [IN_RC_VAS] -> Gain153/1
  Sum32/1 -> Outport5/1, [MN_BFSH]
  [IN_IB_BFSH] -> Gain160/1
  [IN_II_VAS_1] -> Gain158/1
  [IN_RC_BFSH] -> Gain161/1
  [IN_IA_RF] -> Gain156/1
  [SN_IA_BFSH] -> Gain154/1
  [IN_II_BFSH_2] -> Gain157/1
  [IN_IA_VAS] -> Gain155/1
  [IN_II_RF_1] -> Gain159/1
  Sum33/1 -> [MN_GAS], Outport6/1
  [IN_RC_GAS] -> Gain168/1
  [IN_II_TA_1] -> Gain165/1
  [IN_IBext_GAS] -> Gain167/1
  [IN_IB_GAS] -> Gain166/1
  [IN_II_GAS_2] -> Gain164/1
  [SN_IA_GAS] -> Gain162/1
  [IN_IA_TA] -> Gain163/1
  [IN_IA_TA] -> Gain170/1
  [SN_IA_SOL] -> Gain169/1
  [IN_II_SOL_2] -> Gain171/1
  [IN_RC_SOL] -> Gain175/1
  [IN_II_TA_1] -> Gain172/1
  [IN_IBext_SOL] -> Gain174/1
  Sum34/1 -> [MN_SOL], Outport7/1
  [IN_IB_SOL] -> Gain173/1
  Sum35/1 -> Outport8/1, [MN_TA]
  [IN_IB_TA] -> Gain182/1
  [IN_II_GAS_1] -> Gain180/1
  [IN_RC_TA] -> Gain183/1
  [IN_IA_SOL] -> Gain178/1
  [SN_IA_TA] -> Gain176/1
  [IN_II_TA_2] -> Gain179/1
  [IN_IA_GAS] -> Gain177/1
  [IN_II_SOL_1] -> Gain181/1
  [SN_IA_HFL] -> Gain1/1
  [IN_IA_GLU] -> Gain2/1
  [IN_IA_HAM] -> Gain3/1
  [IN_RC_GLU] -> Gain4/1
  [IN_RC_HAM] -> Gain5/1
  [MN_HFL] -> Gain7/1
  [SN_IB_HFL] -> Gain8/1
  [IN_IB_HAM] -> Gain10/1
  [IN_IB_GLU] -> Gain9/1
  [IN_RC_GLU] -> Gain13/1
  [Act_HFL] -> Gain12/1
  [IN_RC_HAM] -> Gain11/1
  Gain1/1 -> Sum1/1  "SNIA HFL"
  Gain2/1 -> Sum1/2  "INIA GLU"
  Gain3/1 -> Sum1/3  "INIA HAM"
  Gain4/1 -> Sum1/4  "INRC GLU"
  Gain7/1 -> Sum1/6  "MN HFL"
  Gain5/1 -> Sum1/5  "INRC HAM"
  Gain10/1 -> Sum4/3
  Gain8/1 -> Sum4/1
  Gain9/1 -> Sum4/2
  Gain13/1 -> Sum5/2
  Gain11/1 -> Sum5/3
  Gain12/1 -> Sum5/1
  Gain16/1 -> Sum/2
  Gain15/1 -> Sum/1
  Gain14/1 -> Sum/3
  Gain17/1 -> Sum/4
  Gain19/1 -> Sum2/1
  Gain20/1 -> Sum2/2
  Gain22/1 -> Sum3/1
  Gain23/1 -> Sum3/2
  Gain24/1 -> Sum6/1
  Gain26/1 -> Sum6/3
  Gain28/1 -> Sum6/5
  Gain25/1 -> Sum6/2
  Gain27/1 -> Sum6/4
  Gain29/1 -> Sum6/6
  Gain31/1 -> Sum7/1
  Gain33/1 -> Sum7/3
  Gain32/1 -> Sum7/2
  Gain35/1 -> Sum8/1
  Gain37/1 -> Sum8/3
  Gain36/1 -> Sum8/2
  Gain40/1 -> Sum9/3
  Gain38/1 -> Sum9/1
  Gain39/1 -> Sum9/2
  Gain41/1 -> Sum9/4
  Gain42/1 -> Sum9/5
  Gain43/1 -> Sum9/6
  Gain46/1 -> Sum10/2
  Gain47/1 -> Sum10/3
  Gain45/1 -> Sum10/1
  Gain49/1 -> Sum11/1
  Gain51/1 -> Sum11/3
  Gain50/1 -> Sum11/2
  Gain54/1 -> Sum14/3
  Gain52/1 -> Sum14/1
  Gain53/1 -> Sum14/2
  Gain55/1 -> Sum14/4
  Gain56/1 -> Sum14/5
  Gain57/1 -> Sum14/6
  Gain60/1 -> Sum12/2
  Gain61/1 -> Sum12/3
  Gain59/1 -> Sum12/1
  Gain64/1 -> Sum13/3
  Gain62/1 -> Sum13/1
  Gain63/1 -> Sum13/2
  Gain66/1 -> Sum15/1
  Gain68/1 -> Sum15/3
  Gain67/1 -> Sum15/2
  Gain69/1 -> Sum15/4
  Gain70/1 -> Sum15/5
  Gain71/1 -> Sum15/6
  Gain73/1 -> Sum16/1
  Gain74/1 -> Sum16/2
  Gain75/1 -> Sum16/3
  Gain77/1 -> Sum17/2
  Gain76/1 -> Sum17/1
  Gain78/1 -> Sum17/3
  Gain79/1 -> Sum18/1  "SN IA GAS"
  Gain81/1 -> Sum18/3  "IN RC TA"
  Gain80/1 -> Sum18/2  "IN IA TA"
  Gain82/1 -> Sum18/4  "MN GAS"
  Gain83/1 -> Saturation116/1  "SN II GAS"
  Gain84/1 -> Sum19/1  "SN IB GAS"
  Gain85/1 -> Sum19/2  "IN IB TA"
  Gain86/1 -> Sum20/1  "ACT GAS"
  Gain87/1 -> Sum20/2  "IN RC TA"
  Gain88/1 -> Saturation118/1  "SN IBEXT GAS"
  Gain91/1 -> Sum21/3  "IN RC TA"
  Gain90/1 -> Sum21/2  "IN IA TA"
  Gain89/1 -> Sum21/1  "SN IA SOL"
  Gain92/1 -> Sum21/4  "MN SOL"
  Gain93/1 -> Saturation121/1  "SN II SOL"
  Gain94/1 -> Sum22/1  "SN IB SOL"
  Gain95/1 -> Sum22/2  "INIB TA"
  Gain96/1 -> Saturation123/1  "SN IB SOL EXT"
  Gain97/1 -> Sum23/1  "ACT SOL"
  Gain98/1 -> Sum23/2  "RC TA"
  Gain99/1 -> Sum24/1  "SNIA TA"
  Gain100/1 -> Sum24/2  "INIA GAS"
  Gain101/1 -> Sum24/3  "INIA SOL"
  Gain103/1 -> Sum24/5  "INRC SOL"
  Gain102/1 -> Sum24/4  "INRC GAS"
  Gain104/1 -> Sum24/6  "MN TA"
  Gain105/1 -> Saturation126/1  "SN II TA"
  Gain107/1 -> Sum25/2  "INIB GAS"
  Gain106/1 -> Sum25/1  "SN IB TA"
  Gain108/1 -> Sum25/3  "INIB SOL"
  Gain110/1 -> Sum26/2  "INRC GAS"
  Gain111/1 -> Sum26/3  "INRC SOL"
  Gain109/1 -> Sum26/1  "ACT TA"
  Gain112/1 -> Sum28/1
  Gain114/1 -> Sum28/3
  Gain113/1 -> Sum28/2
  Gain115/1 -> Sum28/4
  Gain116/1 -> Sum28/5
  Gain117/1 -> Sum28/6
  Gain118/1 -> Sum28/7
  Gain119/1 -> Sum28/8
  Gain120/1 -> Sum27/1
  Gain121/1 -> Sum27/2
  Gain123/1 -> Sum27/4
  Gain122/1 -> Sum27/3
  Gain125/1 -> Sum27/6
  Gain124/1 -> Sum27/5
  Gain126/1 -> Sum27/7
  Gain133/1 -> Sum29/7
  Gain131/1 -> Sum29/5
  Gain134/1 -> Sum29/8
  Gain132/1 -> Sum29/6
  Gain127/1 -> Sum29/1
  Gain129/1 -> Sum29/3
  Gain130/1 -> Sum29/4
  Gain128/1 -> Sum29/2
  Gain135/1 -> Sum29/9
  Gain136/1 -> Sum30/1
  Gain144/1 -> Sum30/9
  Gain142/1 -> Sum30/7
  Gain138/1 -> Sum30/3
  Gain140/1 -> Sum30/5
  Gain139/1 -> Sum30/4
  Gain141/1 -> Sum30/6
  Gain137/1 -> Sum30/2
  Gain143/1 -> Sum30/8
  Gain145/1 -> Sum31/1
  Gain146/1 -> Sum31/2
  Gain147/1 -> Sum31/3
  Gain148/1 -> Sum31/4
  Gain153/1 -> Sum31/9
  Gain149/1 -> Sum31/5
  Gain150/1 -> Sum31/6
  Gain152/1 -> Sum31/8
  Gain151/1 -> Sum31/7
  Gain154/1 -> Sum32/1
  Gain157/1 -> Sum32/4
  Gain155/1 -> Sum32/2
  Gain161/1 -> Sum32/8
  Gain158/1 -> Sum32/5
  Gain156/1 -> Sum32/3
  Gain159/1 -> Sum32/6
  Gain160/1 -> Sum32/7
  Gain168/1 -> Sum33/7
  Gain167/1 -> Sum33/6
  Gain163/1 -> Sum33/2
  Gain162/1 -> Sum33/1
  Gain164/1 -> Sum33/3
  Gain166/1 -> Sum33/5
  Gain165/1 -> Sum33/4
  Gain169/1 -> Sum34/1
  Gain172/1 -> Sum34/4
  Gain175/1 -> Sum34/7
  Gain170/1 -> Sum34/2
  Gain174/1 -> Sum34/6
  Gain173/1 -> Sum34/5
  Gain171/1 -> Sum34/3
  Gain179/1 -> Sum35/4
  Gain177/1 -> Sum35/2
  Gain178/1 -> Sum35/3
  Gain176/1 -> Sum35/1
  Gain183/1 -> Sum35/8
  Gain182/1 -> Sum35/7
  Gain180/1 -> Sum35/5
  Gain181/1 -> Sum35/6
  Sum1/1 -> Saturation87/1
  Gain6/1 -> Saturation88/1, Scope20/1
  Sum4/1 -> Saturation89/1
  Sum5/1 -> Saturation90/1
  Sum/1 -> Saturation91/1
  Gain18/1 -> Saturation92/1
  Sum2/1 -> Saturation93/1
  Gain21/1 -> Saturation94/1
  Sum3/1 -> Saturation95/1
  Sum6/1 -> Saturation96/1
  Gain30/1 -> Saturation97/1
  Sum7/1 -> Saturation98/1
  Gain34/1 -> Saturation99/1
  Sum8/1 -> Saturation100/1
  Sum9/1 -> Saturation101/1
  Gain44/1 -> Saturation102/1
  Sum10/1 -> Saturation103/1
  Gain48/1 -> Saturation104/1
  Sum11/1 -> Saturation105/1
  Sum14/1 -> Saturation106/1
  Gain58/1 -> Saturation107/1
  Sum12/1 -> Saturation108/1
  Gain65/1 -> Saturation109/1
  Sum13/1 -> Saturation110/1
  Sum15/1 -> Saturation111/1
  Gain72/1 -> Saturation112/1
  Sum16/1 -> Saturation113/1
  Sum17/1 -> Saturation114/1
  Sum18/1 -> Saturation115/1
  Sum19/1 -> Saturation117/1
  Sum20/1 -> Saturation119/1
  Sum21/1 -> Saturation120/1
  Sum22/1 -> Saturation122/1
  Sum23/1 -> Saturation124/1
  Sum24/1 -> Saturation125/1
  Sum25/1 -> Saturation127/1
  Sum26/1 -> Saturation128/1
  Saturation51/1 -> [SN_IB_HFL]
  Saturation53/1 -> [SN_IA_HFL]
  Saturation52/1 -> [SN_II_HFL]
  Saturation55/1 -> [SN_II_GLU]
  Saturation54/1 -> [SN_IB_GLU]
  Saturation56/1 -> [SN_IA_GLU]
  Saturation59/1 -> [SN_IA_HAM]
  Saturation57/1 -> [SN_IB_HAM]
  Saturation58/1 -> [SN_II_HAM]
  Saturation60/1 -> [SN_IB_RF]
  Saturation62/1 -> [SN_IA_RF]
  Saturation61/1 -> [SN_II_RF]
  Saturation63/1 -> [SN_IB_VAS]
  Saturation65/1 -> [SN_IA_VAS]
  Saturation64/1 -> [SN_II_VAS]
  Saturation68/1 -> [SN_IA_BFSH]
  Saturation67/1 -> [SN_II_BFSH]
  Saturation66/1 -> [SN_IB_BFSH]
  Saturation71/1 -> [SN_IA_GAS]
  Saturation70/1 -> [SN_II_GAS]
  Saturation69/1 -> [SN_IB_GAS]
  Saturation72/1 -> [SN_IB_SOL]
  Saturation74/1 -> [SN_IA_SOL]
  Saturation73/1 -> [SN_II_SOL]
  Saturation75/1 -> [SN_IB_TA]
  Saturation77/1 -> [SN_IA_TA]
  Saturation76/1 -> [SN_II_TA]
  Saturation47/1 -> [IN_IA_TA]
  Saturation48/1 -> [IN_II_TA_1]
  Saturation49/1 -> [IN_II_TA_2]
  Saturation50/1 -> [IN_IB_TA]
  Saturation78/1 -> [IN_RC_TA]
  Saturation46/1 -> [IN_RC_SOL]
  Saturation42/1 -> [IN_IA_SOL]
  Saturation45/1 -> [IN_IBext_SOL]
  Saturation43/1 -> [IN_II_SOL_1]
  Saturation44/1 -> [IN_IB_SOL]
  Saturation37/1 -> [IN_IA_GAS]
  Saturation38/1 -> [IN_II_GAS_1]
  Saturation39/1 -> [IN_IB_GAS]
  Saturation41/1 -> [IN_RC_GAS]
  Saturation40/1 -> [IN_IBext_GAS]
  Saturation79/1 -> [IN_II_GAS_2]
  Saturation80/1 -> [IN_II_SOL_2]
  Saturation35/1 -> [IN_IB_BFSH]
  Saturation33/1 -> [IN_IA_BFSH]
  Saturation34/1 -> [IN_II_BFSH_1]
  Saturation36/1 -> [IN_RC_BFSH]
  Saturation81/1 -> [IN_II_BFSH_2]
  Saturation29/1 -> [IN_II_VAS_1]
  Saturation28/1 -> [IN_IA_VAS]
  Saturation30/1 -> [IN_IB_VAS]
  Saturation32/1 -> [IN_RC_VAS]
  Saturation31/1 -> [IN_IBext_VAS]
  Saturation82/1 -> [IN_II_VAS_2]
  Saturation25/1 -> [IN_IB_RF]
  Saturation23/1 -> [IN_IA_RF]
  Saturation24/1 -> [IN_II_RF_1]
  Saturation26/1 -> [IN_IBext_RF]
  Saturation27/1 -> [IN_RC_RF]
  Saturation83/1 -> [IN_II_RF_2]
  Saturation22/1 -> [IN_RC_HAM]
  Saturation21/1 -> [IN_IBext_HAM]
  Saturation19/1 -> [IN_II_HAM_1]
  Saturation18/1 -> [IN_IA_HAM]
  Saturation20/1 -> [IN_IB_HAM]
  Saturation84/1 -> [IN_II_HAM_2]
  Saturation15/1 -> [IN_IB_GLU]
  Saturation13/1 -> [IN_IA_GLU]
  Saturation17/1 -> [IN_RC_GLU]
  Saturation14/1 -> [IN_II_GLU_1]
  Saturation16/1 -> [IN_IBext_GLU]
  Saturation85/1 -> [IN_II_GLU_2]
  Saturation10/1 -> [IN_II_HFL_1]
  Saturation11/1 -> [IN_IB_HFL]
  Saturation9/1 -> [IN_IA_HFL]
  Saturation86/1 -> [IN_II_HFL_2]
  Saturation12/1 -> [IN_RC_HFL]
  Saturation87/1 -> IN RC48/1(in)
  Saturation88/1 -> IN RC49/1(in), IN RC50/1(in)
  Saturation89/1 -> IN RC51/1(in)
  Saturation90/1 -> IN RC41/1(in)
  Saturation91/1 -> IN RC42/1(in)
  Saturation92/1 -> IN RC43/1(in), IN RC44/1(in)
  Saturation93/1 -> IN RC45/1(in)
  Saturation94/1 -> IN RC46/1(in)
  Saturation95/1 -> IN RC47/1(in)
  Saturation96/1 -> IN RC35/1(in)
  Saturation97/1 -> IN RC36/1(in), IN RC37/1(in)
  Saturation98/1 -> IN RC38/1(in)
  Saturation99/1 -> IN RC39/1(in)
  Saturation100/1 -> IN RC40/1(in)
  Saturation101/1 -> IN RC29/1(in)
  Saturation102/1 -> IN RC30/1(in), IN RC31/1(in)
  Saturation103/1 -> IN RC32/1(in)
  Saturation104/1 -> IN RC33/1(in)
  Saturation105/1 -> IN RC34/1(in)
  Saturation106/1 -> IN RC23/1(in)
  Saturation107/1 -> IN RC24/1(in), IN RC25/1(in)
  Saturation108/1 -> IN RC26/1(in)
  Saturation109/1 -> IN RC27/1(in)
  Saturation110/1 -> IN RC28/1(in)
  Saturation111/1 -> IN RC18/1(in)
  Saturation112/1 -> IN RC19/1(in), IN RC20/1(in)
  Saturation113/1 -> IN RC21/1(in)
  Saturation114/1 -> IN RC22/1(in)
  Saturation115/1 -> IN RC12/1(in)
  Saturation116/1 -> IN RC13/1(in), IN RC14/1(in)
  Saturation117/1 -> IN RC15/1(in)
  Saturation118/1 -> IN RC16/1(in)
  Saturation119/1 -> IN RC17/1(in)
  Saturation120/1 -> IN RC5/1(in)
  Saturation121/1 -> IN RC6/1(in), IN RC7/1(in)
  Saturation122/1 -> IN RC9/1(in)
  Saturation123/1 -> IN RC10/1(in)
  Saturation124/1 -> IN RC11/1(in)
  Saturation125/1 -> IN RC4/1(in)
  Saturation126/1 -> IN RC3/1(in), IN RC2/1(in)
  Saturation127/1 -> IN RC1/1(in)
  Saturation128/1 -> IN RC8/1(in)

== system nms_sim_2D_cost/CPG-reflex-synergy controller/phi left3 ==
  LStance : Inport
  In1 : Inport  Port=2
  Clock : Clock
  Constant : Constant  Value=omega_4
  Gain : Gain  Gain=gamma_4
  Integrator : Integrator  ExternalReset=rising  InitialConditionSource=external  InitialCondition=init_RCPG
  Pi : Constant  Value=pi  OutDataTypeStr=Inherit: Inherit via back propagation
  Scope : Scope
  Sin : Trigonometry
  Subtract : Sum  Inputs=+--
  Sum : Sum  Inputs=|+-
  Switch : Switch  Criteria=u2 > Threshold  SaturateOnIntegerOverflow=off  InputSameDT=off
  Zero : Constant  Value=0  OutDataTypeStr=Inherit: Inherit via back propagation
  Zero1 : Constant  Value=init_LCPG  OutDataTypeStr=Inherit: Inherit via back propagation
  phi out : Outport
  wires:
  Sin/1 -> Gain/1
  Gain/1 -> Sum/2
  Constant/1 -> Sum/1
  Pi/1 -> Subtract/3
  Subtract/1 -> Sin/1
  Sum/1 -> Integrator/1
  Integrator/1 -> phi out/1, Subtract/1
  In1/1 -> Subtract/2
  LStance/1 -> Integrator/2
  Clock/1 -> Switch/2
  Zero/1 -> Switch/1
  Zero1/1 -> Switch/3
  Switch/1 -> Integrator/3, Scope/1

== system nms_sim_2D_cost/CPG-reflex-synergy controller/phi right ==
  In1 : Inport
  RStance : Inport  Port=2
  Clock : Clock
  Constant : Constant  Value=omega_4
  Gain : Gain  Gain=gamma_4
  Integrator : Integrator  ExternalReset=rising  InitialConditionSource=external  InitialCondition=init_RCPG
  Pi : Constant  Value=pi  OutDataTypeStr=Inherit: Inherit via back propagation
  Scope : Scope
  Sin : Trigonometry
  Subtract : Sum  Inputs=+--
  Sum : Sum  Inputs=|+-
  Switch : Switch  Criteria=u2 > Threshold  SaturateOnIntegerOverflow=off  InputSameDT=off
  Zero : Constant  Value=0  OutDataTypeStr=Inherit: Inherit via back propagation
  Zero1 : Constant  Value=init_RCPG  OutDataTypeStr=Inherit: Inherit via back propagation
  phi out : Outport
  wires:
  Switch/1 -> Scope/1, Integrator/3
  Zero1/1 -> Switch/3
  Zero/1 -> Switch/1
  Clock/1 -> Switch/2
  RStance/1 -> Integrator/2
  In1/1 -> Subtract/2
  Integrator/1 -> Subtract/1, phi out/1
  Sum/1 -> Integrator/1
  Subtract/1 -> Sin/1
  Pi/1 -> Subtract/3
  Constant/1 -> Sum/1
  Gain/1 -> Sum/2
  Sin/1 -> Gain/1

== system nms_sim_2D_cost/Cost/ACT ==
  Mux20 : Mux  Inputs=2
  Mux3 : Mux  Inputs=9
  Mux5 : Mux  Inputs=9
  ACT : Outport
  wires:
  Mux5/1 -> Mux20/2
  Mux3/1 -> Mux20/1
  [RActSOL] -> Mux3/8  "SOL"
  [RActRF] -> Mux3/4  "RF"
  [RActGAS] -> Mux3/7  "GAS"
  [RActTA] -> Mux3/9  "TA"
  [RActBFSH] -> Mux3/6  "BFSH"
  [RActHAM] -> Mux3/3  "HAM"
  [LActGAS] -> Mux5/7  "GAS"
  [LActGLU] -> Mux5/2  "GLU"
  [RActVAS] -> Mux3/5  "VAS"
  [LActTA] -> Mux5/9  "TA"
  [LActVAS] -> Mux5/5  "VAS"
  [RActHFL] -> Mux3/1  "HFL"
  [LActBFSH] -> Mux5/6  "BFSH"
  [LActHAM] -> Mux5/3  "HAM"
  [LActHFL] -> Mux5/1  "HFL"
  [LActSOL] -> Mux5/8  "SOL"
  [RActGLU] -> Mux3/2  "GLU"
  [LActRF] -> Mux5/4  "RF"
  Mux20/1 -> ACT/1

== system nms_sim_2D_cost/Cost/SS_dist ==
  SS_dist : Inport
  Trigger : TriggerPort  VariantControl=Variant  ZeroCross=off
  To Current Workspace4 : ToWorkspace  VariableName=v_SSdist  SaveFormat=Timeseries  SampleTime=-1
      settings: MaxDataPoints=nStep_obj
  wires:
  SS_dist/1 -> To Current Workspace4/1

== system nms_sim_2D_cost/Cost/Step Counter ==
  RStance : Inport
  LStance : Inport  Port=2
  Constant1 : Constant  Value=0
  Constant2 : Constant  Value=0
  Constant3 : Constant  Value=0
  Constant4 : Constant  Value=-1
  Saturation Dynamic : simulink/Discontinuities/Saturation Dynamic  OutMin=[]  OutMax=[]  OutDataTypeStr=Inherit: Same as second input  OutDataType=fixdt(1, 16)  OutScaling=2^-10  DoSatur=off
  Saturation Dynamic1 : simulink/Discontinuities/Saturation Dynamic  OutMin=[]  OutMax=[]  OutDataTypeStr=Inherit: Same as second input  OutDataType=fixdt(1, 16)  OutScaling=2^-10  DoSatur=off
  Sum : Sum  Inputs=|++
  Sum1 : Sum  Inputs=++|
  Sum2 : Sum  Inputs=|++
  count steps1 : Subsystem  TreatAsAtomicUnit=on
  count steps2 : Subsystem  TreatAsAtomicUnit=on
  nStep : Outport
  wires:
  Sum/1 -> nStep/1
  Sum2/1 -> Saturation Dynamic/1  "up lim"
  Constant4/1 -> Sum2/1
  Saturation Dynamic1/1 -> count steps1/1(nStep-1)
  Constant2/1 -> Saturation Dynamic1/3
  Sum1/1 -> Saturation Dynamic1/1
  Constant1/1 -> Sum1/2
  Saturation Dynamic/1 -> count steps2/1(nStep-1)  "output"
  Constant3/1 -> Saturation Dynamic/3
  count steps2/1(nStep) -> Sum/1, Saturation Dynamic/2, Sum1/1  "u"
  count steps1/1(nStep) -> Sum/2, Sum2/2, Saturation Dynamic1/2
  RStance/1 -> count steps2/Trigger
  LStance/1 -> count steps1/Trigger

== system nms_sim_2D_cost/Cost/calculate ObjFn ==
  nStep : Inport
  nStep_start : Inport  Port=2
  ACT : Inport  Port=3
  pain : Inport  Port=4
  flight : Inport  Port=5
  x : Inport  Port=6
  t [s] : Inport  Port=7
  Enable : EnablePort  ZeroCross=off
  Constant : Constant  Value=nStep_obj
  Relational Operator : RelationalOperator  Operator=>  OutDataTypeStr=boolean  ZeroCross=off  InputSameDT=off
  Relational Operator1 : RelationalOperator  Operator=>  OutDataTypeStr=boolean  ZeroCross=off  InputSameDT=off
  Sum : Sum  Inputs=++|
  calculate A^n : Subsystem  TreatAsAtomicUnit=on
  calculate flight : Subsystem  TreatAsAtomicUnit=on
  calculate pain : Subsystem  TreatAsAtomicUnit=on
  start flight : Subsystem  TreatAsAtomicUnit=on
  startA2 : Subsystem  TreatAsAtomicUnit=on
  startPain : Subsystem  TreatAsAtomicUnit=on
  startPos : Subsystem  TreatAsAtomicUnit=on
  startTime : Subsystem  TreatAsAtomicUnit=on
  update data : Subsystem  TreatAsAtomicUnit=on
  stop : Outport
  wires:
  startA2/1(A^n_0) -> update data/1(ACT2_0)
  ACT/1 -> calculate A^n/1(A)
  Sum/1 -> Relational Operator1/2
  update data/1(stop) -> stop/1
  nStep/1 -> Relational Operator/1, Relational Operator1/1
  Relational Operator/1 -> calculate A^n/Enable, startA2/Trigger, startPain/Trigger, calculate pain/Enable, startPos/Trigger, startTime/Trigger, start flight/Trigger, calculate flight/Enable
  calculate A^n/1(A^n) -> update data/2(ACT2_1), startA2/1(A^n)
  Relational Operator1/1 -> update data/Enable
  Constant/1 -> Sum/1
  nStep_start/1 -> Sum/2, Relational Operator/2
  startPos/1(x_0) -> update data/7(hipP_0)
  x/1 -> update data/8(hipP_1), startPos/1(x)
  t [s]/1 -> update data/10(t_1), startTime/1(t)
  startTime/1(t_0) -> update data/9(t_0)
  startPain/1(pain_0) -> update data/3(pain_0)
  pain/1 -> calculate pain/1(P)
  calculate pain/1(P_all) -> update data/4(P_all), startPain/1(pain)
  start flight/1(F_0) -> update data/5(F_0)
  calculate flight/1(F_int) -> update data/6(F_int), start flight/1(F)
  flight/1 -> calculate flight/1(F)

== system nms_sim_2D_cost/Cost/check steady state ==
  p : Inport
  nStep : Inport  Port=2
  Abs : Abs  ZeroCross=off  SaturateOnIntegerOverflow=off
  Add{,1..9} (10 alike) : Sum  Inputs=-+
  Add{10..14} (5 alike) : Sum  Inputs=+-
  Compare To Constant : simulink/Logic and Bit Operations/Compare To Constant  relop=>  const=nStep_startKin  OutDataTypeStr=boolean
  Constant7 : Constant  Value=SSW_kin
  Constant8 : Constant  Value=0
  Demux1 : Demux  Outputs=6
  Demux2 : Demux  Outputs=6
  Demux3 : Demux  Outputs=6
  Fcn : Fcn  Expr=rem(u(1), 2)
  Logical Operator : Logic  AllPortsSameDT=off  OutDataTypeStr=boolean
  Mux1 : Mux  Inputs=5
  Mux17 : Mux  Inputs=6
  Relational Operator : RelationalOperator  Operator=<=  OutDataTypeStr=boolean  ZeroCross=off  InputSameDT=off
  Sum of Elements : Sum  Inputs=+
  Switch : Switch  Criteria=u2 > Threshold  Threshold=nStep_startKin  ZeroCross=off  SaturateOnIntegerOverflow=off  InputSameDT=off
  even : Subsystem  TreatAsAtomicUnit=on
  odd : Subsystem  TreatAsAtomicUnit=on
  SS : Outport
  SS_dist : Outport  Port=2
  wires:
  nStep/1 -> Fcn/1, Compare To Constant/1, Switch/2
  Add8/1 -> Add13/2
  Demux2/3 -> Add1/2
  Sum of Elements/1 -> Relational Operator/1, SS_dist/1
  Compare To Constant/1 -> Logical Operator/2
  Constant7/1 -> Switch/1
  Add2/1 -> Add12/1
  Demux1/1 -> Mux17/5
  Demux1/4 -> Mux17/4
  Add5/1 -> Add10/2
  Mux17/1 -> even/1(In1)
  Demux3/4 -> Add7/2
  Abs/1 -> Sum of Elements/1
  Demux1/3 -> Mux17/3
  p/1 -> odd/1(In1), Demux1/1
  Switch/1 -> Relational Operator/2
  Relational Operator/1 -> Logical Operator/1
  Demux2/4 -> Add2/2
  Demux3/1 -> Add5/1, Add6/1, Add7/1, Add8/1, Add9/1
  odd/1(Out1) -> Demux2/1
  Add4/1 -> Add14/1
  Constant8/1 -> Switch/3
  Add/1 -> Add10/1
  Demux1/5 -> Mux17/1
  Demux1/2 -> Mux17/6
  Demux2/1 -> Add/1, Add1/1, Add2/1, Add3/1, Add4/1
  Logical Operator/1 -> SS/1
  Add7/1 -> Add12/2
  Add1/1 -> Add11/1
  Demux3/5 -> Add8/2
  Demux3/3 -> Add6/2
  Add6/1 -> Add11/2
  Add12/1 -> Mux1/3
  Demux2/5 -> Add3/2
  Demux1/6 -> Mux17/2
  Demux3/2 -> Add5/2
  Demux2/2 -> Add/2
  even/1(Out1) -> Demux3/1
  Add13/1 -> Mux1/4
  Add10/1 -> Mux1/1
  Fcn/1 -> odd/Trigger, even/Trigger
  Add11/1 -> Mux1/2
  Add3/1 -> Add13/1
  Add9/1 -> Add14/2
  Mux1/1 -> Abs/1
  Demux3/6 -> Add9/2
  Demux2/6 -> Add4/2
  Add14/1 -> Mux1/5

== system nms_sim_2D_cost/Cost/flight ==
  Max : MinMax  Function=max  Inputs=2
  Minus : Sum  Inputs=+-
  One : Constant  OutDataTypeStr=Inherit: Inherit via back propagation
  flight : Outport
  wires:
  [LStance] -> Max/2  "LStance"
  [RStance] -> Max/1  "RStance"
  Minus/1 -> flight/1
  One/1 -> Minus/1
  Max/1 -> Minus/2
